simulink model "DQstatcom3p"  (R2025a)
settings: Solver=ode23tb  StartTime=0.0  StopTime=0.2  FixedStep=1e-6  MaxStep=1e-6  RelTol=1e-3  EnableMultiTasking=on
undefined symbols (not defined in the file): Vsrc_LL
libraries: spsCurrentMeasurementLib x7, spsMosfetLib x6, spsVoltageMeasurementLib x5, spsSeriesRLCBranchLib x4, powerlib_extras x3, spsThreePhaseParallelRLCLoadLib x1, spsThreePhaseSourceLib x1, spspowerguiLib x1
settings Model: Creator=Rajesh  LastModifiedBy=SimuVerity Contributors
settings SolverCC: ZeroCrossControl=DisableAll  AlgebraicLoopSolver=TrustRegion  SolverResetMethod=Robust
settings DataIOCC: SaveFormat=Array  SignalLoggingSaveFormat=ModelDataLogs  SaveOutput=off  SignalLogging=off  DSMLogging=off  SaveTime=off  ReturnWorkspaceOutputs=off
settings OptimizationCC: ExpressionDepthLimit=2147483647.0  LifeSpan=inf
settings DebuggingCC: UnderspecifiedInitializationDetection=Classic  MergeDetectMultiDrivingBlocksExec=none  SolverPrmCheckMsg=warning  FcnCallInpInsideContextMsg=warning  UnconnectedInputMsg=warning  UnconnectedOutputMsg=warning  UnconnectedLineMsg=warning  StateNameClashWarn=warning  SFUnexpectedBacktrackingDiag=warning  SFNoUnconditionalDefaultTransitionDiag=warning  SFExecutionAtInitializationDiag=none  ArithmeticOperatorsInVariantConditions=warning
settings HardwareCC: ProdBitPerPointer=32.0  ProdBitPerSizeT=32.0  ProdBitPerPtrDiffT=32.0  ProdLargestAtomicFloat=None  ProdIntDivRoundTo=Undefined  ProdEndianess=Unspecified  ProdWordSize=32.0  ProdHWDeviceType=32-bit Generic
settings ModelReferenceCC: EnableRefExpFcnMdlSchedulingChecks=on  PropagateSignalLabelsOutOfModel=off
settings SFSimCC: SimUseLocalCustomCode=off  CustomCodeUndefinedFunction=UseInterfaceOnly
settings RTWCC: RTWUseLocalCustomCode=off  GPUComputeCapability=3.5
settings CodeAppCC: StateflowObjectComments=on
settings GRTTargetCC: TargetLangStandard=C89/C90 (ANSI)  CombineOutputUpdateFcns=off  GRTInterface=on
settings ConfigComp: CovMetricSettings=dw  CovSaveCumulativeToWorkspaceVar=on  CovSaveSingleToWorkspaceVar=on  CovExternalEMLEnable=off
settings SimscapeCC: SimscapeNormalizeSystem=off

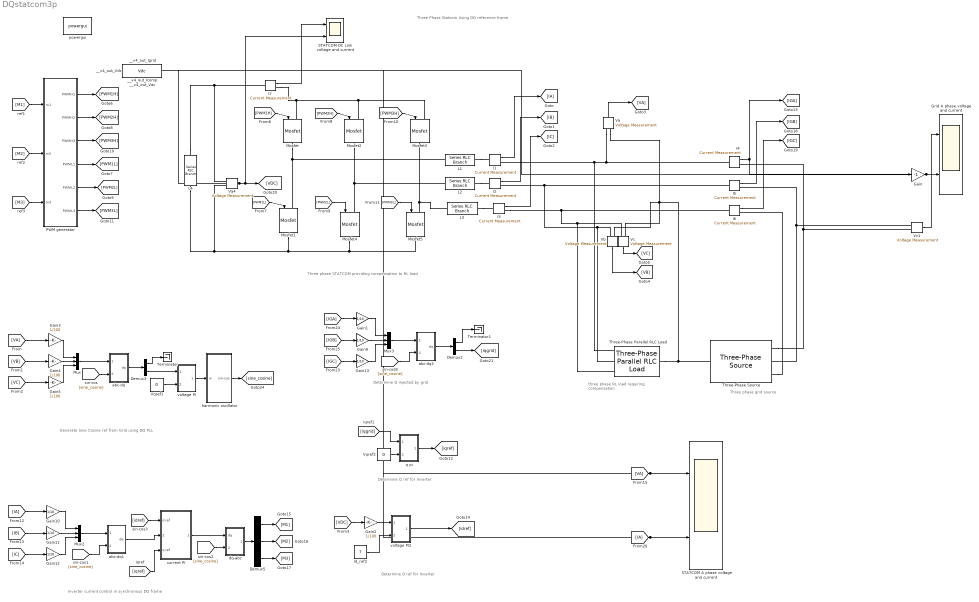
== system DQstatcom3p ==
  note: Inverter current control in synchronous DQ frame
  note: Generate Sine Cosine ref from Grid using DQ PLL
  note: Determine D ref for Inverter
  note: Determine Q ref for Inverter
  note: Determine Q injected by grid
  note: Three phase STATCOM providing compensation to RL load
  note: Three phase grid source
  note: three phase RL load requiring compensation
  note: Three Phase Statcom Using DQ reference frame
  Demux2 : Demux  Outputs=2
  Demux3 : Demux  Outputs=2
  Demux5 : Demux  Outputs=3
  Gain : Gain  Gain=-1
  Gain{1,9..13} (6 alike) : Gain  Gain=1/10
  Gain{2..5} (4 alike) : Gain  Gain=1/100
  Grid A phase voltage and current : Scope  NumInputPorts=2
      settings: ActiveDisplayYMinimum=-416.17914  ActiveDisplayYMaximum=417.53953  DataLoggingMaxPoints=10000  DataLoggingVariableName=ScopeData2
  I{1..7} (7 alike) : spsCurrentMeasurementLib/Current Measurement  PhasorSimulation=off  OutputType=Complex  PSBequivalent=0
  Id_ref2 : Constant  Value=7
  L1 : spsSeriesRLCBranchLib/Series RLC Branch  LConnTagsString=__new0  RConnTagsString=__new0  BranchType=L  Resistance=1.5  Inductance=3e-3  SetiL0=off  InitialCurrent=0  Capacitance=1e-6  Setx0=off  InitialVoltage=0  Measurements=None
  L2 : spsSeriesRLCBranchLib/Series RLC Branch  LConnTagsString=__new0  RConnTagsString=__new0  BranchType=L  Resistance=1.5  Inductance=3e-3  SetiL0=off  InitialCurrent=0  Capacitance=1e-6  Setx0=off  InitialVoltage=0  Measurements=None
  L3 : spsSeriesRLCBranchLib/Series RLC Branch  LConnTagsString=__new0  RConnTagsString=__new0  BranchType=L  Resistance=1.5  Inductance=3e-3  SetiL0=off  InitialCurrent=0  Capacitance=1e-6  Setx0=off  InitialVoltage=0  Measurements=None
  L4 : spsSeriesRLCBranchLib/Series RLC Branch  LConnTagsString=__new0  RConnTagsString=__new0  BranchType=C  Resistance=1.5  Inductance=2.5e-3  SetiL0=off  InitialCurrent=0  Capacitance=10000e-6  Setx0=on  InitialVoltage=700  Measurements=None
  Mosfet{,1..5} (6 alike) : spsMosfetLib/Mosfet  Ron=0.1  Lon=0  Rd=0.01  Vfd=1  IC=0  Rs=1e5  Cs=inf  Measurements=off
  Mux : Mux  Inputs=3
  Mux2 : Mux  Inputs=3
  Mux3 : Mux  Inputs=3
  PWM generator : Subsystem
  STATCOM A phase voltage and current : Scope  NumInputPorts=2
      settings: ActiveDisplayYMinimum=-342.66058  ActiveDisplayYMaximum=255.89373  DataLoggingMaxPoints=10000
  STATCOM DC Link voltage and current : Scope  NumInputPorts=2
      settings: ActiveDisplayYMinimum=-227.29409  ActiveDisplayYMaximum=271.19322  DataLoggingMaxPoints=10000  DataLoggingVariableName=ScopeData9
  Terminator : Terminator
  Terminator1 : Terminator
  Three-Phase Parallel RLC Load : spsThreePhaseParallelRLCLoadLib/Three-Phase Parallel RLC Load  LConnTagsString=A|B|C  RConnTagsString=N  Configuration=Y (neutral)  NominalVoltage=400  Vabc=[1e3 1e3 1e3]  Vabcp=[1e3 1e3 1e3]  NominalFrequency=50  UnbalancedPower=off  ActivePower=P_load  InductivePower=10000  CapacitivePower=0  Pabc=[10e3 9e3 11e3]  QLabc=[100 90 110]  QCabc=[100 90 110]  Pabcp=[10e3 9e3 11e3]  QLabcp=[100 90 110]  QCabcp=[100 90 110]  Measurements=None  LoadType=constant Z
  Three-Phase Source : spsThreePhaseSourceLib/Three-Phase Source  InternalConnection=Yn  VoltagePhases=off  Voltage=Vsrc_LL  PhaseAngle=0  Voltage_phases=[25e3 25e3 25e3]/sqrt(3)  PhaseAngles_phases=[0 -120 +120]  Frequency=50  NonIdealSource=on  SpecifyImpedance=on  Resistance=1e-3  Inductance=1e-3  ShortCircuitLevel=1e6  BaseVoltage=1e3  XRratio=7  BusType=swing  Pref=0  Qref=0  Prefabc=[10e3, 10e3, 10e3]  Qrefabc=[0, 0, 0]  Qmin=-inf  Qmax=inf
  Va : spsVoltageMeasurementLib/Voltage Measurement  PhasorSimulation=off  OutputType=Complex  PSBequivalent=0
  Va4 : spsVoltageMeasurementLib/Voltage Measurement  PhasorSimulation=off  OutputType=Complex  PSBequivalent=0
  Vb : spsVoltageMeasurementLib/Voltage Measurement  PhasorSimulation=off  OutputType=Complex  PSBequivalent=0
  Vc : spsVoltageMeasurementLib/Voltage Measurement  PhasorSimulation=off  OutputType=Complex  PSBequivalent=0
  Vc1 : spsVoltageMeasurementLib/Voltage Measurement  PhasorSimulation=off  OutputType=Complex  PSBequivalent=0
  Vqref1 : Constant  Value=0
  Vqref2 : Constant  Value=0
  __v4_out_Icomp : ToWorkspace  VariableName=Icomp  SaveFormat=Timeseries  SampleTime=-1
  __v4_out_Igrid : ToWorkspace  VariableName=Igrid  SaveFormat=Timeseries  SampleTime=-1
  __v4_out_Vac : ToWorkspace  VariableName=Vac  SaveFormat=Timeseries  SampleTime=-1
  __v4_out_Vdc : ToWorkspace  VariableName=Vdc  SaveFormat=Timeseries  SampleTime=-1
  abc-dq : Subsystem
  abc-dq1 : Subsystem
  abc-dq3 : Subsystem
  current PI : Subsystem
  dq-abc : Subsystem
  harmonic oscillator : Subsystem
  powergui : spspowerguiLib/powergui  Priority=1  SimulationMode=Continuous  SampleTime=50e-6  frequency=60  Iterations=50  frequencyindice=0  Pbase=100e6  ErrMax=1e-4  UnitsV=kV  UnitsW=MW  buscounter=0  FunctionMessages=off  echomessages=off  EnableUseOfTLC=off  CurrentSourceSwitches=off  DisableSnubberDevices=off  DisableRonSwitches=off  DisableVfSwitches=off  DisplayEquations=off  AutomaticDiscreteSolvers=off  SolverType=Tustin  Interpol=off  ExternalGateDelay=off  methode=off  Ts=100  x0status=blocks  SPID=off  SwTol=0  HookPort=off  NonlinearTolerance=1e-4  nMaxIteration=100  ContinueOnMaxIteration=off  RestoreLinks=warning  ResistiveCurrentMeasurement=off  Frange=[0:2:500]  Ylog=off  Xlog=on  ShowGrid=off  save=off  variable=ZData  structure=0  ZoomFFT=off  StartTime=0.0  cycles=1  DisplayStyle=1  fundamental=60  FreqAxis=off  MaxFrequency=1000  frequencyindicesteady=1  RmsSteady=1  display=off
  q pi : Subsystem
  voltage PI : Subsystem
  voltage PI2 : Subsystem
  wires:
  I3/1 -> [IC]
  I2/1 -> [IB]
  I1/1 -> [IA]
  Va/1 -> [VA]
  Vc/1 -> [VC]
  Vb/1 -> [VB]
  [VA] -> Gain3/1
  [VB] -> Gain4/1
  [VC] -> Gain5/1
  Gain4/1 -> Mux/2
  Gain3/1 -> Mux/1
  Gain5/1 -> Mux/3
  Mux/1 -> abc-dq/1(abc)
  harmonic oscillator/1(sin-cos) -> [sine_cosine]
  abc-dq/1(dq) -> Demux3/1
  [IA] -> Gain10/1
  [IB] -> Gain11/1
  [IC] -> Gain12/1
  Gain11/1 -> Mux2/2
  Gain10/1 -> Mux2/1
  Gain12/1 -> Mux2/3
  I7/1 -> STATCOM DC Link voltage and current/1
  Demux3/2 -> voltage PI/1(q in)
  PWM generator/1(PWMH1) -> [PWM1H]
  PWM generator/2(PWMH2) -> [PWM2H]
  PWM generator/3(PWMH3) -> [PWM3H]
  PWM generator/4(PWML1) -> [PWM1L]
  PWM generator/5(PWML2) -> [PWM2L]
  PWM generator/6(PWML3) -> [PWM3L]
  [M1] -> PWM generator/1(m1)
  [M2] -> PWM generator/2(m2)
  [M3] -> PWM generator/3(m3)
  voltage PI/1(w out) -> harmonic oscillator/1(w)
  Vqref1/1 -> voltage PI/2(q ref)
  [sine_cosine] -> abc-dq/2(sin-cos)
  Mux2/1 -> abc-dq1/1(abc)
  [sine_cosine] -> abc-dq1/2(sin-cos)
  abc-dq1/1(dq) -> current PI/2(dq pi in)
  current PI/1(dq pi out) -> dq-abc/1(dq)
  [sine_cosine] -> dq-abc/2(sin-cos)
  Demux5/1 -> [M1]
  Demux5/2 -> [M2]
  Demux5/3 -> [M3]
  Va4/1 -> [VDC], STATCOM DC Link voltage and current/2, __v4_out_Vdc/1
  dq-abc/1(abc) -> Demux5/1
  [PWM1H] -> Mosfet/1
  [PWM2H] -> Mosfet2/1
  [PWM3H] -> Mosfet3/1
  [PWM1L] -> Mosfet1/1
  [PWM2L] -> Mosfet4/1
  [PWM3L] -> Mosfet5/1
  [VDC] -> Gain2/1
  Id_ref2/1 -> voltage PI2/2(Vdc ref)
  [idref] -> current PI/1(d ref)
  Demux3/1 -> Terminator/1
  I6/1 -> [IGC]
  I5/1 -> [IGB]
  voltage PI2/1(Idref) -> [idref]
  [IGA] -> Gain1/1
  [IGB] -> Gain9/1
  [IGC] -> Gain13/1
  Gain9/1 -> Mux3/2
  Gain1/1 -> Mux3/1
  Gain13/1 -> Mux3/3
  Mux3/1 -> abc-dq3/1(abc)
  [sine_cosine] -> abc-dq3/2(sin-cos)
  abc-dq3/1(dq) -> Demux2/1
  Demux2/2 -> [iqgrid]
  [VA] -> STATCOM A phase voltage and current/1, __v4_out_Vac/1
  Vqref2/1 -> q pi/2(Iq ref)
  q pi/1(Iq out) -> [iqref]
  [iqgrid] -> q pi/1(Iq in)
  Gain2/1 -> voltage PI2/1(Vdc in)
  Demux2/1 -> Terminator1/1
  Gain/1 -> Grid A phase voltage and current/2, __v4_out_Igrid/1
  Vc1/1 -> Grid A phase voltage and current/1
  I4/1 -> [IGA], Gain/1
  [IA] -> STATCOM A phase voltage and current/2, __v4_out_Icomp/1
  [iqref] -> current PI/3(q ref)
  connections:
  L1/RConn1 -- I1/LConn1
  L2/RConn1 -- I2/LConn1
  L3/RConn1 -- I3/LConn1
  Mosfet/RConn1 -- Mosfet1/LConn1 -- L1/LConn1
  Mosfet2/RConn1 -- Mosfet4/LConn1 -- L2/LConn1
  Mosfet5/LConn1 -- Mosfet3/RConn1 -- L3/LConn1
  L4/RConn1 -- Mosfet5/RConn1 -- Mosfet4/RConn1 -- Mosfet1/RConn1 -- Va4/LConn2
  Mosfet3/LConn1 -- Mosfet2/LConn1 -- Mosfet/LConn1 -- I7/RConn1
  L4/LConn1 -- I7/LConn1 -- Va4/LConn1
  Three-Phase Source/RConn1 -- I4/RConn1 -- Vc1/LConn1
  Three-Phase Source/RConn3 -- I6/RConn1
  Three-Phase Source/LConn1 -- Vb/LConn2 -- Vc/LConn2 -- Va/LConn2 -- Three-Phase Parallel RLC Load/RConn1
  Vc/LConn1 -- Three-Phase Parallel RLC Load/LConn3 -- I6/LConn1 -- I3/RConn1
  Vb/LConn1 -- I5/LConn1 -- I2/RConn1 -- Three-Phase Parallel RLC Load/LConn2
  Va/LConn1 -- I4/LConn1 -- I1/RConn1 -- Three-Phase Parallel RLC Load/LConn1
  Vc1/LConn2 -- Three-Phase Source/RConn2 -- I5/RConn1

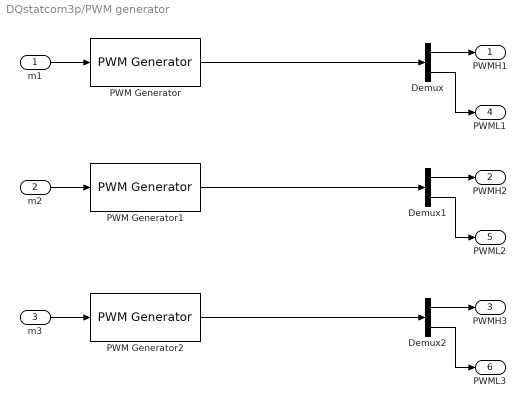
== system DQstatcom3p/PWM generator ==
  m1 : Inport
  m2 : Inport  Port=2
  m3 : Inport  Port=3
  Demux : Demux  Outputs=2
  Demux1 : Demux  Outputs=2
  Demux2 : Demux  Outputs=2
  PWM Generator : powerlib_extras/Control  Blocks/PWM Generator  GeneratorMode="1-arm  bridge (2 pulses)"  Fc=7500  Internal=off  mIndex=0.4  Freq=60  Phase=0
  PWM Generator1 : powerlib_extras/Control  Blocks/PWM Generator  GeneratorMode="1-arm  bridge (2 pulses)"  Fc=7500  Internal=off  mIndex=0.4  Freq=60  Phase=0
  PWM Generator2 : powerlib_extras/Control  Blocks/PWM Generator  GeneratorMode="1-arm  bridge (2 pulses)"  Fc=7500  Internal=off  mIndex=0.4  Freq=60  Phase=0
  PWMH1 : Outport  VectorParamsAs1DForOutWhenUnconnected=off
  PWMH2 : Outport  Port=2  VectorParamsAs1DForOutWhenUnconnected=off
  PWMH3 : Outport  Port=3  VectorParamsAs1DForOutWhenUnconnected=off
  PWML1 : Outport  Port=4  VectorParamsAs1DForOutWhenUnconnected=off
  PWML2 : Outport  Port=5  VectorParamsAs1DForOutWhenUnconnected=off
  PWML3 : Outport  Port=6  VectorParamsAs1DForOutWhenUnconnected=off
  wires:
  Demux2/2 -> PWML3/1
  Demux2/1 -> PWMH3/1
  Demux1/2 -> PWML2/1
  Demux1/1 -> PWMH2/1
  Demux/2 -> PWML1/1
  Demux/1 -> PWMH1/1
  m1/1 -> PWM Generator/1
  m2/1 -> PWM Generator1/1
  m3/1 -> PWM Generator2/1
  PWM Generator/1 -> Demux/1
  PWM Generator1/1 -> Demux1/1
  PWM Generator2/1 -> Demux2/1

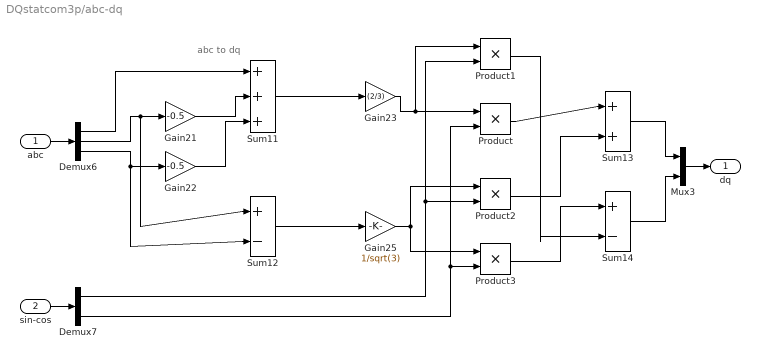
== system DQstatcom3p/abc-dq ==
  note: abc to dq
  abc : Inport
  sin-cos : Inport  Port=2
  Demux6 : Demux  Outputs=3
  Demux7 : Demux  Outputs=2
  Gain21 : Gain  Gain=-0.5
  Gain22 : Gain  Gain=-0.5
  Gain23 : Gain  Gain=(2/3)
  Gain25 : Gain  Gain=1/sqrt(3)
  Mux3 : Mux  Inputs=2
  Product{,1..3} (4 alike) : Product  RndMeth=Zero
  Sum11 : Sum  Inputs=|+++
  Sum12 : Sum  Inputs=|+-
  Sum13 : Sum  Inputs=|++
  Sum14 : Sum  Inputs=|+-
  dq : Outport  VectorParamsAs1DForOutWhenUnconnected=off
  wires:
  Sum11/1 -> Gain23/1
  Sum12/1 -> Gain25/1
  Demux6/3 -> Gain22/1, Sum12/2
  Demux6/2 -> Gain21/1, Sum12/1
  Demux6/1 -> Sum11/1
  Gain21/1 -> Sum11/2
  Gain22/1 -> Sum11/3
  Gain23/1 -> Product/1, Product1/1
  Demux7/2 -> Product/2, Product3/2
  Demux7/1 -> Product1/2, Product2/2
  Gain25/1 -> Product2/1, Product3/1
  Product/1 -> Sum13/1
  Product2/1 -> Sum13/2
  Product3/1 -> Sum14/1
  Product1/1 -> Sum14/2
  Sum13/1 -> Mux3/1
  Sum14/1 -> Mux3/2
  abc/1 -> Demux6/1
  Mux3/1 -> dq/1
  sin-cos/1 -> Demux7/1

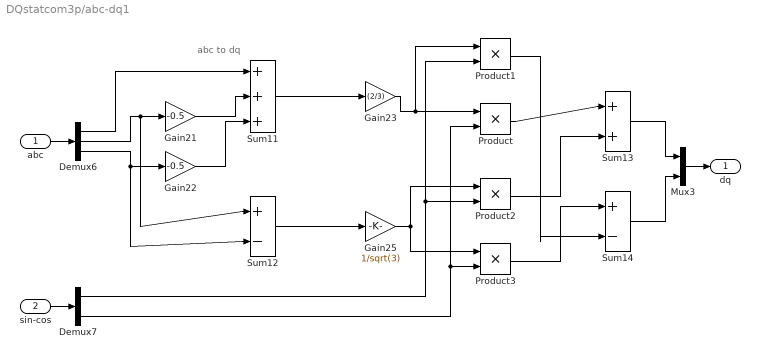
== system DQstatcom3p/abc-dq1 ==
  note: abc to dq
  abc : Inport
  sin-cos : Inport  Port=2
  Demux6 : Demux  Outputs=3
  Demux7 : Demux  Outputs=2
  Gain21 : Gain  Gain=-0.5
  Gain22 : Gain  Gain=-0.5
  Gain23 : Gain  Gain=(2/3)
  Gain25 : Gain  Gain=1/sqrt(3)
  Mux3 : Mux  Inputs=2
  Product{,1..3} (4 alike) : Product  RndMeth=Zero
  Sum11 : Sum  Inputs=|+++
  Sum12 : Sum  Inputs=|+-
  Sum13 : Sum  Inputs=|++
  Sum14 : Sum  Inputs=|+-
  dq : Outport  VectorParamsAs1DForOutWhenUnconnected=off
  wires:
  Sum11/1 -> Gain23/1
  Sum12/1 -> Gain25/1
  Demux6/3 -> Gain22/1, Sum12/2
  Demux6/2 -> Gain21/1, Sum12/1
  Demux6/1 -> Sum11/1
  Gain21/1 -> Sum11/2
  Gain22/1 -> Sum11/3
  Gain23/1 -> Product/1, Product1/1
  Demux7/2 -> Product/2, Product3/2
  Demux7/1 -> Product1/2, Product2/2
  Gain25/1 -> Product2/1, Product3/1
  Product/1 -> Sum13/1
  Product2/1 -> Sum13/2
  Product3/1 -> Sum14/1
  Product1/1 -> Sum14/2
  Sum13/1 -> Mux3/1
  Sum14/1 -> Mux3/2
  abc/1 -> Demux6/1
  Mux3/1 -> dq/1
  sin-cos/1 -> Demux7/1

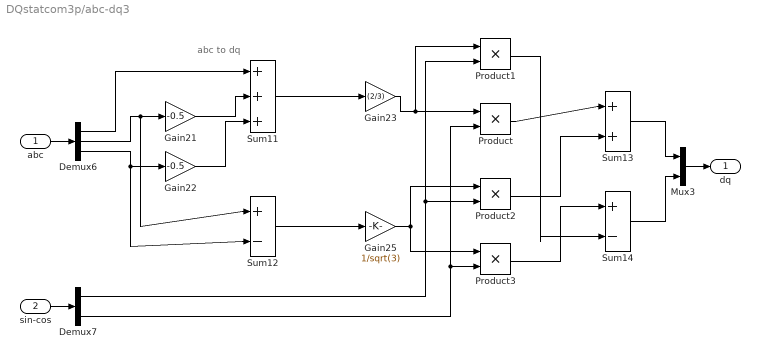
== system DQstatcom3p/abc-dq3 ==
  note: abc to dq
  abc : Inport
  sin-cos : Inport  Port=2
  Demux6 : Demux  Outputs=3
  Demux7 : Demux  Outputs=2
  Gain21 : Gain  Gain=-0.5
  Gain22 : Gain  Gain=-0.5
  Gain23 : Gain  Gain=(2/3)
  Gain25 : Gain  Gain=1/sqrt(3)
  Mux3 : Mux  Inputs=2
  Product{,1..3} (4 alike) : Product  RndMeth=Zero
  Sum11 : Sum  Inputs=|+++
  Sum12 : Sum  Inputs=|+-
  Sum13 : Sum  Inputs=|++
  Sum14 : Sum  Inputs=|+-
  dq : Outport  VectorParamsAs1DForOutWhenUnconnected=off
  wires:
  Sum11/1 -> Gain23/1
  Sum12/1 -> Gain25/1
  Demux6/3 -> Gain22/1, Sum12/2
  Demux6/2 -> Gain21/1, Sum12/1
  Demux6/1 -> Sum11/1
  Gain21/1 -> Sum11/2
  Gain22/1 -> Sum11/3
  Gain23/1 -> Product/1, Product1/1
  Demux7/2 -> Product/2, Product3/2
  Demux7/1 -> Product1/2, Product2/2
  Gain25/1 -> Product2/1, Product3/1
  Product/1 -> Sum13/1
  Product2/1 -> Sum13/2
  Product3/1 -> Sum14/1
  Product1/1 -> Sum14/2
  Sum13/1 -> Mux3/1
  Sum14/1 -> Mux3/2
  abc/1 -> Demux6/1
  Mux3/1 -> dq/1
  sin-cos/1 -> Demux7/1

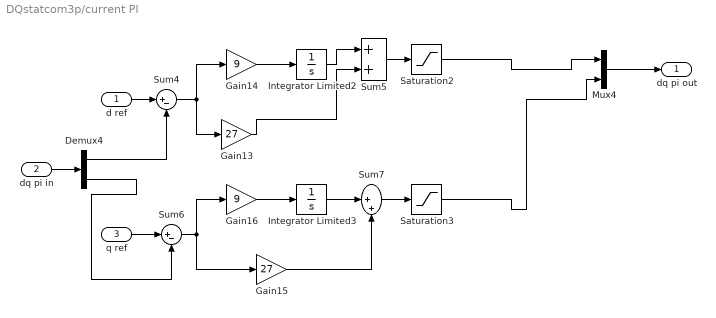
== system DQstatcom3p/current PI ==
  d ref : Inport
  dq pi in : Inport  Port=2
  q ref : Inport  Port=3
  Demux4 : Demux  Outputs=2
  Gain13 : Gain  Gain=27
  Gain14 : Gain  Gain=9
  Gain15 : Gain  Gain=27
  Gain16 : Gain  Gain=9
  Integrator Limited2 : Integrator  LimitOutput=on  UpperSaturationLimit=5  LowerSaturationLimit=-5  ZeroCross=off
  Integrator Limited3 : Integrator  LimitOutput=on  UpperSaturationLimit=5  LowerSaturationLimit=-5  ZeroCross=off
  Mux4 : Mux  Inputs=2
  Saturation2 : Saturate  UpperLimit=5  LowerLimit=-5  ZeroCross=off
  Saturation3 : Saturate  UpperLimit=5  LowerLimit=-5  ZeroCross=off
  Sum4 : Sum  Inputs=|+-
  Sum5 : Sum  Inputs=|++
  Sum6 : Sum  Inputs=|+-
  Sum7 : Sum  Inputs=|++
  dq pi out : Outport  VectorParamsAs1DForOutWhenUnconnected=off
  wires:
  Gain14/1 -> Integrator Limited2/1
  Sum4/1 -> Gain13/1, Gain14/1
  Gain16/1 -> Integrator Limited3/1
  Sum6/1 -> Gain16/1, Gain15/1
  Integrator Limited3/1 -> Sum7/1
  Gain15/1 -> Sum7/2
  Sum5/1 -> Saturation2/1
  Integrator Limited2/1 -> Sum5/1
  Gain13/1 -> Sum5/2
  Mux4/1 -> dq pi out/1
  d ref/1 -> Sum4/1
  dq pi in/1 -> Demux4/1
  Demux4/1 -> Sum4/2
  Saturation3/1 -> Mux4/2
  Saturation2/1 -> Mux4/1
  Sum7/1 -> Saturation3/1
  q ref/1 -> Sum6/1
  Demux4/2 -> Sum6/2

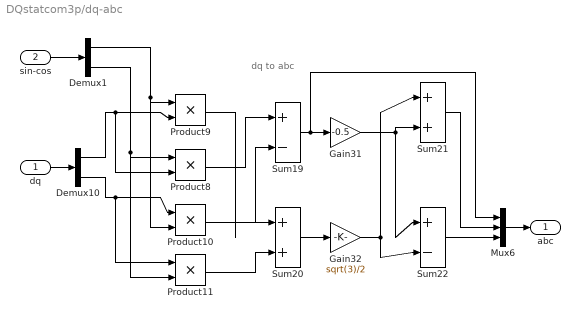
== system DQstatcom3p/dq-abc ==
  note: dq to abc
  dq : Inport
  sin-cos : Inport  Port=2
  Demux1 : Demux  Outputs=2
  Demux10 : Demux  Outputs=2
  Gain31 : Gain  Gain=-0.5
  Gain32 : Gain  Gain=sqrt(3)/2
  Mux6 : Mux  Inputs=3
  Product{8..11} (4 alike) : Product  RndMeth=Zero
  Sum19 : Sum  Inputs=|+-
  Sum20 : Sum  Inputs=|++
  Sum21 : Sum  Inputs=|++
  Sum22 : Sum  Inputs=|+-
  abc : Outport  VectorParamsAs1DForOutWhenUnconnected=off
  wires:
  Sum22/1 -> Mux6/3
  Sum21/1 -> Mux6/2
  Demux10/2 -> Product10/1, Product11/1
  Demux10/1 -> Product9/2, Product8/2
  Gain31/1 -> Sum21/2, Sum22/1
  Gain32/1 -> Sum21/1, Sum22/2
  Sum19/1 -> Gain31/1, Mux6/1
  Sum20/1 -> Gain32/1
  Product10/1 -> Sum19/2
  Product11/1 -> Sum20/2
  Product9/1 -> Sum20/1
  Product8/1 -> Sum19/1
  Demux1/1 -> Product10/2, Product9/1
  Demux1/2 -> Product11/2, Product8/1
  dq/1 -> Demux10/1
  Mux6/1 -> abc/1
  sin-cos/1 -> Demux1/1

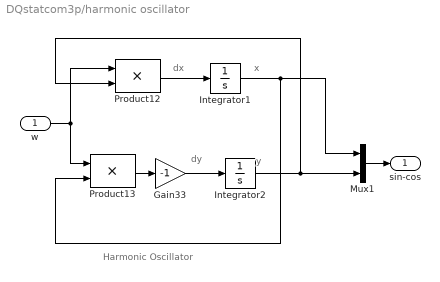
== system DQstatcom3p/harmonic oscillator ==
  note: Harmonic Oscillator
  note: dy
  note: dx
  note: y
  note: x
  w : Inport
  Gain33 : Gain  Gain=-1  SaturateOnIntegerOverflow=on  OutDataTypeStr=Inherit: Same as input  ParamDataTypeStr=Inherit: Same as input
  Integrator1 : Integrator  InitialCondition=1  LimitOutput=on  UpperSaturationLimit=1  LowerSaturationLimit=-1
  Integrator2 : Integrator  LimitOutput=on  UpperSaturationLimit=1  LowerSaturationLimit=-1
  Mux1 : Mux  Inputs=2
  Product12 : Product  SaturateOnIntegerOverflow=on  OutDataTypeStr=Inherit: Same as first input
  Product13 : Product  SaturateOnIntegerOverflow=on  OutDataTypeStr=Inherit: Same as first input
  sin-cos : Outport  VectorParamsAs1DForOutWhenUnconnected=off
  wires:
  w/1 -> Product13/1, Product12/1
  Gain33/1 -> Integrator2/1
  Product12/1 -> Integrator1/1
  Product13/1 -> Gain33/1
  Integrator1/1 -> Product13/2, Mux1/1
  Integrator2/1 -> Product12/2, Mux1/2
  Mux1/1 -> sin-cos/1

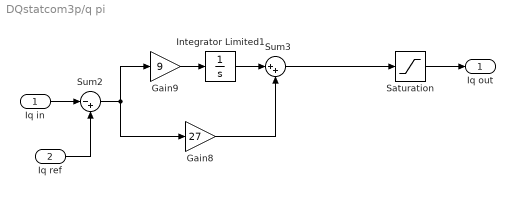
== system DQstatcom3p/q pi ==
  Iq in : Inport
  Iq ref : Inport  Port=2
  Gain8 : Gain  Gain=27
  Gain9 : Gain  Gain=9
  Integrator Limited1 : Integrator  LimitOutput=on  UpperSaturationLimit=314*3  LowerSaturationLimit=-314*3  ZeroCross=off
  Saturation : Saturate  UpperLimit=5  LowerLimit=-5
  Sum2 : Sum  Inputs=|-+
  Sum3 : Sum  Inputs=|++
  Iq out : Outport  VectorParamsAs1DForOutWhenUnconnected=off
  wires:
  Gain8/1 -> Sum3/2
  Integrator Limited1/1 -> Sum3/1
  Sum2/1 -> Gain9/1, Gain8/1
  Gain9/1 -> Integrator Limited1/1
  Iq ref/1 -> Sum2/2
  Iq in/1 -> Sum2/1
  Saturation/1 -> Iq out/1
  Sum3/1 -> Saturation/1

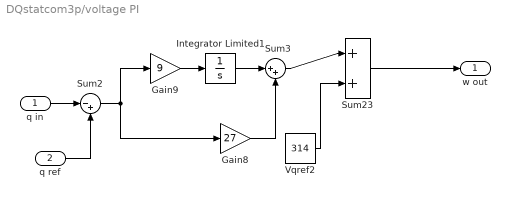
== system DQstatcom3p/voltage PI ==
  q in : Inport
  q ref : Inport  Port=2
  Gain8 : Gain  Gain=27
  Gain9 : Gain  Gain=9
  Integrator Limited1 : Integrator  LimitOutput=on  UpperSaturationLimit=314*3  LowerSaturationLimit=-314*3  ZeroCross=off
  Sum2 : Sum  Inputs=|-+
  Sum23 : Sum  Inputs=|++
  Sum3 : Sum  Inputs=|++
  Vqref2 : Constant  Value=314
  w out : Outport  VectorParamsAs1DForOutWhenUnconnected=off
  wires:
  Vqref2/1 -> Sum23/2
  Gain8/1 -> Sum3/2
  Integrator Limited1/1 -> Sum3/1
  Sum2/1 -> Gain9/1, Gain8/1
  Gain9/1 -> Integrator Limited1/1
  q ref/1 -> Sum2/2
  Sum3/1 -> Sum23/1
  q in/1 -> Sum2/1
  Sum23/1 -> w out/1

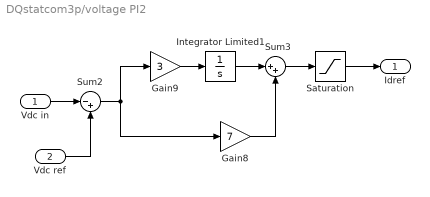
== system DQstatcom3p/voltage PI2 ==
  Vdc in : Inport
  Vdc ref : Inport  Port=2
  Gain8 : Gain  Gain=7
  Gain9 : Gain  Gain=3
  Integrator Limited1 : Integrator  LimitOutput=on  UpperSaturationLimit=314*3  LowerSaturationLimit=-314*3  ZeroCross=off
  Saturation : Saturate
  Sum2 : Sum  Inputs=|-+
  Sum3 : Sum  Inputs=|++
  Idref : Outport  VectorParamsAs1DForOutWhenUnconnected=off
  wires:
  Gain8/1 -> Sum3/2
  Integrator Limited1/1 -> Sum3/1
  Sum2/1 -> Gain9/1, Gain8/1
  Gain9/1 -> Integrator Limited1/1
  Vdc ref/1 -> Sum2/2
  Vdc in/1 -> Sum2/1
  Saturation/1 -> Idref/1
  Sum3/1 -> Saturation/1
